simulink model "Main_with_GuiG"  (R2025b)
settings: Solver=VariableStepAuto  StartTime=0.0  StopTime=10.0  RelTol=1e-3
libraries: SignalEditorBlockLib x2, simulink x2, sharedTrackingLibrary x1, sim3dlib x1, uavsim3dlib x1, sensorgpslib x1, aerolibnav x1
settings Model: Creator=amirs  LastModifiedBy=amirs

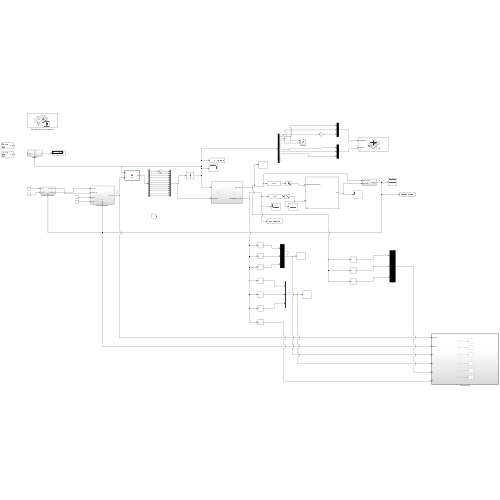
[thumbnail: Simulink's stored preview of the top-level diagram]
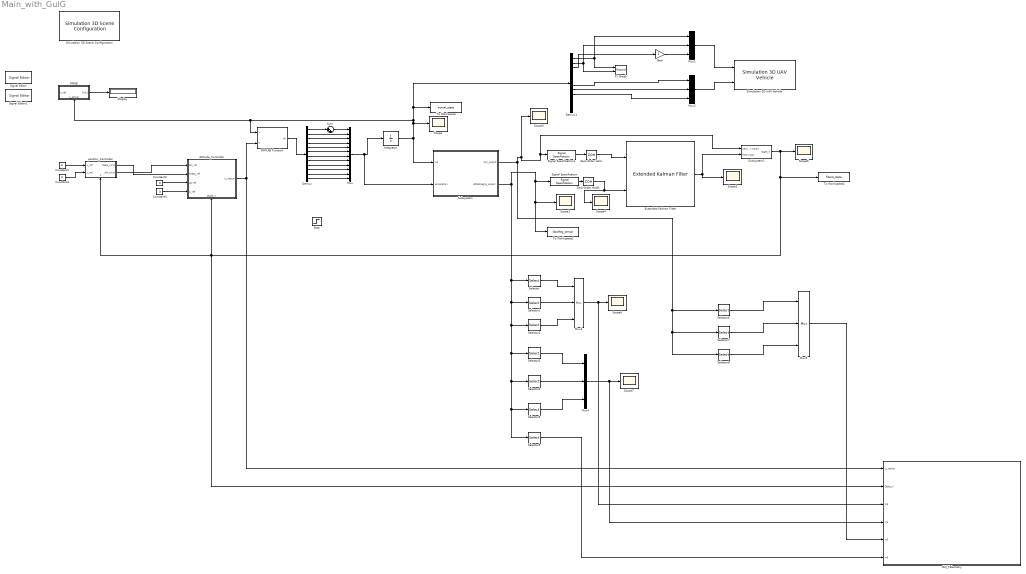
== system Main_with_GuiG ==
  Attitude_Controller : Subsystem
      settings: PortSchema="{\"entries\":[{\"content\":{\"sides\":[{\"content\":{\"connectorIds\":[\"In1\",\"In2\",\"In3\",\"In4\"]},\"type\":\"ConnectorPlacement.EquallySpacedRectSide\",\"uuid\":\"19f4eeea-d5cb-4ed7-9c59-67184399f9de\"},{\"content\":{\"connectorIds\":[\"Out1\"],\"side\":\"RIGHT\"},\"type\":\"ConnectorPlacement.EquallySpacedRectSide\",\"uuid\":\"b3f5ec5c-a38f-4295-9bcf-0fae3bfa674b\"},{\"content\":{\"side\":\"TOP\"},\"type\":\"ConnectorPlacement.EquallySpacedRectSide\",\"uuid\":\"2fc47e81-4ab5-4bbe-b029-56bfdcdb6174\"},{\"content\":{\"connectorIds\":[\"In5\"],\"side\":\"BOTTOM\"},\"type\":\"ConnectorPlacement.EquallySpacedRectSide\",\"uuid\":\"a7c3fd73-d82a-467d-bca9-1f7d01263d9c\"}]},\"type\":\"ConnectorPlacement.EquallySpacedConnector\",\"uuid\":\"700c1ad5-606a-4180-bf9f-c597a2a2a5d4\"}],\"packageUris\":[\"http://schema.mathworks.com/mf0/Connector/R2020b\"],\"version\":\"1.0\"}"
  Constant1 : Constant  Value=3
  Constant2 : Constant  Value=0
  Constant3 : Constant  Value=3
  Constant4 : Constant  Value=2
  Demux : Demux  Outputs=12
  Demux1 : Demux  Outputs=12
  Display : Display
  Extended Kalman Filter : sharedTrackingLibrary/Extended Kalman Filter  StateTransitionFcn=ekfStateTransition  HasStateTransitionJacobianFcn=off  HasAdditiveProcessNoise=Additive  ProcessNoise="[1e-5 1e-5 1e-5  1e-2 1e-2 1e-2  1.5e-6 1.5e-6 1.5e-6]"  HasTimeVaryingProcessNoise=off  HasStateTransitionFcnExtraArgument=1  InitialState=[0,0,0,0,0,0,0,0,0]  InitialStateCovariance=[6.25 6.25 0.04 2.5e-3 2.5e-3 2.5e-3 3e-3 3e-3 1.2e-3]  MeasurementFcn1=ekfMeasurement  HasMeasurementJacobianFcn1=off  HasMeasurementEnablePort1=off  HasAdditiveMeasurementNoise1=Additive  MeasurementNoise1="diag([6.25  7  0.04   2.5e-3  2.5e-3  2.5e-3   1.2e-3])"  HasTimeVaryingMeasurementNoise1=off  HasMeasurementFcnExtraArgument1=0  HasMeasurementWrapping1=off  MeasurementFcn2=ekfMeasTilt  HasMeasurementJacobianFcn2=off  HasMeasurementEnablePort2=off  HasAdditiveMeasurementNoise2=Additive  MeasurementNoise2=diag([2.5e-4 2.5e-4])  HasTimeVaryingMeasurementNoise2=off  HasMeasurementFcnExtraArgument2=0  HasMeasurementWrapping2=off  MeasurementFcn3=myMeasurementFcn  HasMeasurementJacobianFcn3=off  HasMeasurementEnablePort3=off  HasAdditiveMeasurementNoise3=Additive  MeasurementNoise3=1  HasTimeVaryingMeasurementNoise3=off  HasMeasurementFcnExtraArgument3=0  HasMeasurementWrapping3=off  MeasurementFcn4=myMeasurementFcn  HasMeasurementJacobianFcn4=off  HasMeasurementEnablePort4=off  HasAdditiveMeasurementNoise4=Additive  MeasurementNoise4=1  HasTimeVaryingMeasurementNoise4=off  HasMeasurementFcnExtraArgument4=0  HasMeasurementWrapping4=off  MeasurementFcn5=myMeasurementFcn  HasMeasurementJacobianFcn5=off  HasMeasurementEnablePort5=off  HasAdditiveMeasurementNoise5=Additive  MeasurementNoise5=1  HasTimeVaryingMeasurementNoise5=off  HasMeasurementFcnExtraArgument5=0  HasMeasurementWrapping5=off  EnableMultirate=on  StateTransitionFcnSampleTime=0.005  MeasurementFcn1SampleTime=0.1  MeasurementFcn2SampleTime=0.005  MeasurementFcn3SampleTime=1  MeasurementFcn4SampleTime=1  MeasurementFcn5SampleTime=1  UseCurrentEstimator=off  OutputStateCovariance=off  DataType=double  SampleTime=1  NumberOfMeasurements=1
  GUI_Telemetry : Subsystem  TreatAsAtomicUnit=on
  Gain : Gain
  Integrator : Integrator  InitialCondition=[0;0;0;0;0;0;0;0;0;0;0;0]
  MATLAB Function : MATLAB Function  TreatAsAtomicUnit=on
  Mux : Mux  Inputs=12
  Mux{1..5} (5 alike) : Mux  Inputs=3
  RMSE : Subsystem
      settings: PortSchema="{\"entries\":[{\"content\":{\"sides\":[{\"content\":{\"connectorIds\":[\"In1\"]},\"type\":\"ConnectorPlacement.EquallySpacedRectSide\",\"uuid\":\"5e07c89f-ef09-4b0a-bed5-e0d03eb8d545\"},{\"content\":{\"connectorIds\":[\"Out1\"],\"side\":\"RIGHT\"},\"type\":\"ConnectorPlacement.EquallySpacedRectSide\",\"uuid\":\"9156e923-85eb-42fc-9dec-5f08a3c9d42c\"},{\"content\":{\"side\":\"TOP\"},\"type\":\"ConnectorPlacement.EquallySpacedRectSide\",\"uuid\":\"e2ee007b-856b-4d03-8afd-b743321baf7d\"},{\"content\":{\"connectorIds\":[\"In2\"],\"side\":\"BOTTOM\"},\"type\":\"ConnectorPlacement.EquallySpacedRectSide\",\"uuid\":\"3aca7e9a-13ba-49c1-8015-1f7d41362bc4\"}]},\"type\":\"ConnectorPlacement.EquallySpacedConnector\",\"uuid\":\"905e6a99-45d0-4759-a1dd-bed499fabe76\"}],\"packageUris\":[\"http://schema.mathworks.com/mf0/Connector/R2020b\"],\"version\":\"1.0\"}"
  Scope{,1..7} (8 alike) : Scope
      Scope settings: ActiveDisplayYMinimum=-0.58911175900886825  ActiveDisplayYMaximum=5.302005831079815
      Scope1 settings: ActiveDisplayYMinimum=-13.326141979899816  ActiveDisplayYMaximum=19.254724347414861
      Scope2 settings: ActiveDisplayYMinimum=-0.53363237481390613  ActiveDisplayYMaximum=4.8026913733251559  DataLoggingVariableName=ScopeData2
      Scope3 settings: ActiveDisplayYMinimum=-7.8319587540170037  ActiveDisplayYMaximum=0.35536866604481165  DataLoggingVariableName=ScopeData5
      Scope4 settings: ActiveDisplayYMinimum=-7.5918797397091611  ActiveDisplayYMaximum=10.762543329699707  DataLoggingVariableName=ScopeData7
      Scope5 settings: ActiveDisplayYMinimum=-1.7341932188779878  ActiveDisplayYMaximum=7.0655008286033389  DataLoggingVariableName=ScopeData8
      Scope6 settings: ActiveDisplayYMinimum=-7.5918797397091611  ActiveDisplayYMaximum=10.762543329699707  DataLoggingVariableName=ScopeData10
      Scope7 settings: ActiveDisplayYMinimum=-7.5918797397091611  ActiveDisplayYMaximum=10.762543329699707  DataLoggingVariableName=ScopeData11
  Selector : Selector  InputPortWidth=7  IndexOptions=Index vector (dialog)  Indices=[1]  OutputSizes=1
  Selector1 : Selector  InputPortWidth=7  IndexOptions=Index vector (dialog)  Indices=[2]  OutputSizes=1
  Selector2 : Selector  InputPortWidth=7  IndexOptions=Index vector (dialog)  Indices=[3]  OutputSizes=1
  Selector3 : Selector  InputPortWidth=7  IndexOptions=Index vector (dialog)  Indices=[4]  OutputSizes=1
  Selector4 : Selector  InputPortWidth=7  IndexOptions=Index vector (dialog)  Indices=[5]  OutputSizes=1
  Selector5 : Selector  InputPortWidth=7  IndexOptions=Index vector (dialog)  Indices=[6]  OutputSizes=1
  Selector6 : Selector  InputPortWidth=6  IndexOptions=Index vector (dialog)  Indices=[1]  OutputSizes=1
  Selector7 : Selector  InputPortWidth=6  IndexOptions=Index vector (dialog)  Indices=[2]  OutputSizes=1
  Selector8 : Selector  InputPortWidth=6  IndexOptions=Index vector (dialog)  Indices=[3]  OutputSizes=1
  Selector9 : Selector  InputPortWidth=7  IndexOptions=Index vector (dialog)  Indices=[7]  OutputSizes=1
  Signal Editor : SignalEditorBlockLib/Signal Editor  FileName=squer.mat  ActiveScenario=Scenario  ActiveSignal=x_ref  IsBus=off  OutputBusObjectStr=Bus: BusObject  SampleTime=0  ZeroCross=off  OutputAfterFinalValue=Setting to zero  Unit=inherit  PreserveSignalName=on  ApplySigPropsToAllScenarios=on  ApplySigPropsToAllSignals=off  SignalPropertySource=Dialog parameters
  Signal Editor1 : SignalEditorBlockLib/Signal Editor  FileName=squer_y.mat  ActiveScenario=Scenario  ActiveSignal=y_ref  IsBus=off  OutputBusObjectStr=Bus: BusObject  SampleTime=0  ZeroCross=off  OutputAfterFinalValue=Setting to zero  Unit=inherit  PreserveSignalName=on  ApplySigPropsToAllScenarios=on  ApplySigPropsToAllSignals=off  SignalPropertySource=Dialog parameters
  Signal Specification : SignalSpecification  Dimensions=[7]
  Signal Specification1 : SignalSpecification
  Simulation 3D Scene Configuration : sim3dlib/Simulation 3D Scene Configuration  Priority=0  ProjectFormat=Default Scenes  SceneDesc=US city block  ProjectName=C:\Program Files\MATLAB\R2025b\toolbox\shared\sim3d_projects\automotive_project_windows\UE\WindowsNoEditor\VehicleSimulation.exe  ScenePath=/Game/Maps/USCityBlock  EnableOpenDRIVE=off  vehTagList={'Custom';'Scene Origin'}  vehTag=Scene Origin  AttachedCameraRelativeTranslation=[0 0 0]  FreeCameraDefaultInitialTranslation=[-6, 0, 2]  AttachedCameraRelativeRotation=[0 0 0]  FreeCameraDefaultInitialRotation=[0, -15, 0]  ViewpointName=Custom  FreeCameraInitialTranslation=[0, 0, 0]  ViewpointTranslation=[0, 0, 0]  FreeCameraInitialRotation=[0, 0, 0]  ViewpointRotation=[0, 0, 0]  OpVisEn=off  Ts=1/60  EnableWindow=on  EnableRemoteAccess=off  EnableWeather=off  SunAzimuth=90  SunAltitude=40.0  EnableGeospatialSun=off  Latitude=0  Longitude=0  Date=2023-01-01  Time=10:30:00  GeoTimeZone=-5.0  SunDaylightSaving=off  wind=1  clouds=10  EnableVolumetricClouds=off  CloudCoverage=0  CloudAltitude=6  fog=0  rain=0  RaindropsEffect=off  SnowDensity=0  EnableGeospatial=off  TilesetSource=Earth terrain  UseTrueOrigin=off  OriginHeight=200  OriginLatitude=40.744652  OriginLongitude=-73.988864  MapStyle=Aerial  AdditionalAssetIDs=[]  UseAdvancedSunSky=off  SolarTime=11  TimeZone=-5  Day=21  Month=9  Year=2022  UseDaylightSavingTime=on  DSTStartDay=10  DSTStartMonth=3  DSTEndDay=3  DSTEndMonth=11  DSTSwitchHour=2  sensorTag=MainCamera1  sensorId=1  sensorName=MainCamera1  mountLoc=Origin  offsetFlag=off  tmountOffset=[0, 0, 0]  rmountOffset=[0, 0, 0]  HorizontalResolution=1280  VerticalResolution=720  HorizontalFOV=60  mountPoint=[0 0 0]  mountOrientation=[0 0 0]  aMode=4  ID=1  GeoTrigger=Inactive  ViewNameList={'Custom'}  ViewTranslationList={'[0 0 0]'}  ViewRotationList={'[0 0 0]'}
      settings: LibrarySourceBlock=uavsim3dlib/Simulation 3D Scene Configuration
  Simulation 3D UAV Vehicle : uavsim3dlib/Simulation 3D UAV Vehicle  Priority=-1  Mesh=Quadrotor  MeshPath=/MathWorksUAVContent/UAVs/HexaRotorUAV/HexaRotor.HexaRotor  Color=Green  ActorName=SimulinkVehicle1  UseGlobalFrame=off  InitialTranslation=[0 0 0]  InitialRotation=[0 0 0]  InitialTranslationGlobal=[0 0 0]  InitialGeoOrigin=[0 0 0]  InitialRotationGlobal=[0 0 0]  SampleTime=-1  ActorType=SimulinkVehicle  ID=1  aMode=4  ActorTag=SimulinkVehicle1
  Step : Step  Time=25  After=0  SampleTime=0
  Subsystem : Subsystem
  Subsystem1 : Subsystem
  Sum : Sum  Inputs=|++
  To Workspace : ToWorkspace  VariableName=actual_state  SampleTime=-1
      settings: Save2DSignal=2-D array (concatenate along first dimension)
  To Workspace1 : ToWorkspace  VariableName=GpsMag_sensor  SampleTime=-1
      settings: Save2DSignal=2-D array (concatenate along first dimension)
  To Workspace2 : ToWorkspace  VariableName=filterd_state  SampleTime=-1
      settings: Save2DSignal=2-D array (concatenate along first dimension)
  XY Graph : Record  NumPorts=2.0  FileSettingsInternal="{\"entries\":[{\"content\":{\"excelSettings\":{\"content\":{},\"type\":\"Streamout.ExcelSettings\"},\"parquetSettings\":{\"content\":{},\"type\":\"Streamout.ParquetSettings\"}},\"type\":\"Streamout.FileSettingStorage\",\"uuid\":\"\"}],\"packageUris\":[\"http:\\/\\/schema.mathworks.com\\/mf0\\/streamout_blocks\\/R2020a\"],\"version\":\"1.0\"}"  FrameSettings=[0, 0]  Layout=[1 1]  SignalsInternal="{\"entries\":[{\"content\":{\"signals\":[{\"content\":{\"blockPath\":[],\"dimensions\":[1],\"domain\":\"\",\"lineColor\":\"#64d413\",\"lineWidth\":2,\"port\":1,\"sid\":[\"\"],\"signalID\":1,\"signalName\":\"Demux1:1\"},\"type\":\"RecordBlkView.Signal\",\"uuid\":\"\"},{\"content\":{\"blockPath\":[],\"dimensions\":[1],\"domain\":\"\",\"lineColor\":\"#ff13a6\",\"lineWidth\":2,\"port\":2,\"sid\":[\"\"],\"signalID\":2,\"signalName\":\"Demux1:2\"},\"type\":\"RecordBlkView.Signal\",\"uuid\":\"\"}]},\"type\":\"RecordBlkView.InputSignals\",\"uuid\":\"\"}],\"packageUris\":[\"http:\\/\\/schema.mathworks.com\\/mf0\\/streamout_blocks\\/R2020a\"],\"version\":\"1.0\"}"  VisualizationBindings="{\"xyplotplugin\":{\"info\":[{\"series\":[],\"subplotID\":1}]}}"  CompatibilityTag=XY
  Zero-Order Hold : ZeroOrderHold  SampleTime=0.005
  Zero-Order Hold1 : ZeroOrderHold  SampleTime=0.1
  position_Controller : Subsystem
      settings: PortSchema="{\"entries\":[{\"content\":{\"sides\":[{\"content\":{\"connectorIds\":[\"In1\",\"In2\"]},\"type\":\"ConnectorPlacement.EquallySpacedRectSide\",\"uuid\":\"b3fdc6c0-3d6b-4fed-ba04-72ee8971ce33\"},{\"content\":{\"connectorIds\":[\"Out1\",\"Out2\"],\"side\":\"RIGHT\"},\"type\":\"ConnectorPlacement.EquallySpacedRectSide\",\"uuid\":\"c5fff90f-3f0d-4e66-bfd3-42639056edf5\"},{\"content\":{\"side\":\"TOP\"},\"type\":\"ConnectorPlacement.EquallySpacedRectSide\",\"uuid\":\"29c618c7-b581-4d0e-90c8-5996712070e8\"},{\"content\":{\"connectorIds\":[\"In3\"],\"side\":\"BOTTOM\"},\"type\":\"ConnectorPlacement.EquallySpacedRectSide\",\"uuid\":\"80cb8360-5186-4b4a-b3bf-580e229b7937\"}]},\"type\":\"ConnectorPlacement.EquallySpacedConnector\",\"uuid\":\"86696893-c9ee-41ff-bf75-cf6f558ac07e\"}],\"packageUris\":[\"http://schema.mathworks.com/mf0/Connector/R2020b\"],\"version\":\"1.0\"}"
  wires:
  Demux/12 -> Mux/12
  Demux/6 -> Mux/6
  Sum/1 -> Mux/1
  Mux/1 -> Subsystem/2(accleration), Integrator/1
  Demux/1 -> Sum/1
  RMSE/1(Out1) -> Display/1
  Gain/1 -> Mux1/3
  position_Controller/1(theta_cmd) -> Attitude_Controller/2(Theta_ref)
  Extended Kalman Filter/1 -> Subsystem1/2(filter input), Scope2/1
  Demux/5 -> Mux/5
  Subsystem/2(GPS&Magno_output) -> To Workspace1/1, Scope1/1, Signal Specification/1, Selector4/1, Selector9/1, Selector5/1, Selector3/1, Selector2/1, Selector1/1, Selector/1
  Demux/4 -> Mux/4
  Integrator/1 -> Subsystem/1(In1), Scope/1, To Workspace/1, Demux1/1, MATLAB Function/1(X), RMSE/2(x_actual)
  Demux/9 -> Mux/9
  Demux/11 -> Mux/11
  Zero-Order Hold/1 -> Extended Kalman Filter/1
  Demux1/2 -> XY Graph/2, Mux1/2
  Subsystem1/1(State_X) -> To Workspace2/1, GUI_Telemetry/2(State_X), position_Controller/3(X), Attitude_Controller/5(State_X), Scope5/1
  Demux/3 -> Mux/3
  Demux/2 -> Mux/2
  Demux1/7 -> Mux2/1
  Constant1/1 -> position_Controller/1(x_ref)
  position_Controller/2(phi_cmd) -> Attitude_Controller/1(phi_ref)
  Demux1/8 -> Mux2/2
  Demux1/9 -> Mux2/3
  Signal Specification/1 -> Zero-Order Hold1/1
  Constant3/1 -> Attitude_Controller/4(Z_ref)
  Demux1/1 -> Mux1/1, XY Graph/1
  Zero-Order Hold1/1 -> Extended Kalman Filter/2, Scope4/1
  Demux1/3 -> Gain/1
  Demux/8 -> Mux/8
  Mux2/1 -> Simulation 3D UAV Vehicle/2
  Demux/10 -> Mux/10
  Signal Specification1/1 -> Zero-Order Hold/1
  Demux/7 -> Mux/7
  Attitude_Controller/1(U_vector) -> MATLAB Function/2(U), GUI_Telemetry/1(U_vector)
  MATLAB Function/1(dX) -> Demux/1
  Constant2/1 -> Attitude_Controller/3(psi ref)
  Mux1/1 -> Simulation 3D UAV Vehicle/1
  Constant4/1 -> position_Controller/2(y_ref)
  Selector/1 -> Mux3/1
  Selector1/1 -> Mux3/2
  Selector2/1 -> Mux3/3
  Mux3/1 -> GUI_Telemetry/3(In3), Scope6/1
  Selector3/1 -> Mux4/1
  Selector4/1 -> Mux4/2
  Selector5/1 -> Mux4/3
  Mux4/1 -> GUI_Telemetry/4(In4), Scope7/1
  Subsystem/1(IMU_output) -> Subsystem1/1(sensor input1), Signal Specification1/1, Scope3/1, Selector8/1, Selector7/1, Selector6/1
  Selector7/1 -> Mux5/2
  Selector8/1 -> Mux5/3
  Selector6/1 -> Mux5/1
  Mux5/1 -> GUI_Telemetry/5(In5)
  Selector9/1 -> GUI_Telemetry/6(In6)

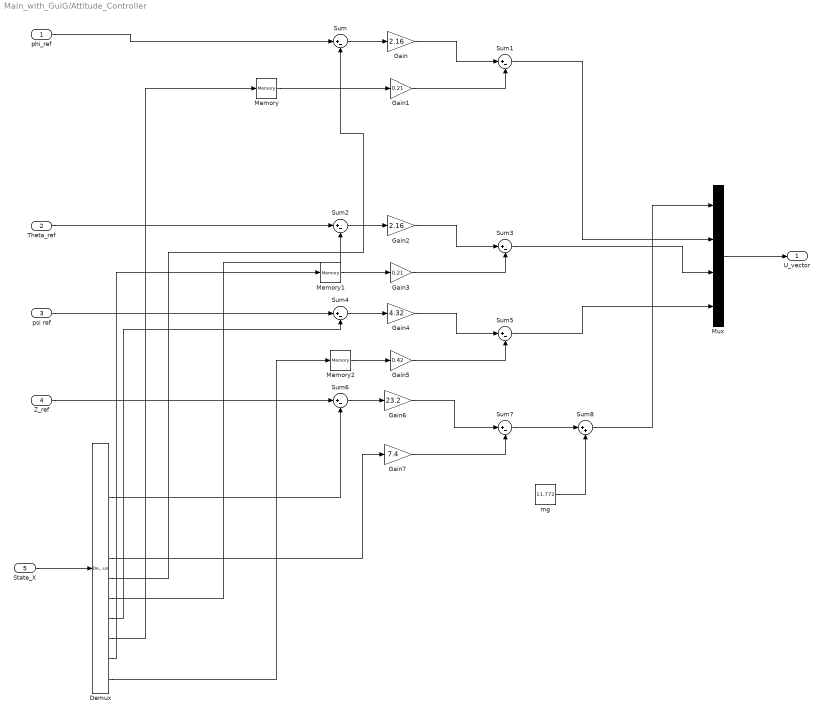
== system Main_with_GuiG/Attitude_Controller ==
  phi_ref : Inport
  Theta_ref : Inport  Port=2
  psi ref : Inport  Port=3
  Z_ref : Inport  Port=4
  State_X : Inport  Port=5
  Demux : Demux  Outputs=12
  Gain : Gain  Gain=2.16
  Gain1 : Gain  Gain=0.21
  Gain2 : Gain  Gain=2.16
  Gain3 : Gain  Gain=0.21
  Gain4 : Gain  Gain=4.32
  Gain5 : Gain  Gain=0.42
  Gain6 : Gain  Gain=23.2
  Gain7 : Gain  Gain=7.4
  Memory : Memory
  Memory1 : Memory
  Memory2 : Memory
  Mux : Mux
  Sum{,1..7} (8 alike) : Sum  Inputs=|+-
  Sum8 : Sum  Inputs=|++
  mg : Constant  Value=11.772
  U_vector : Outport
  wires:
  State_X/1 -> Demux/1
  phi_ref/1 -> Sum/1
  Demux/7 -> Sum/2
  Sum/1 -> Gain/1
  Gain/1 -> Sum1/1
  Gain1/1 -> Sum1/2
  Gain3/1 -> Sum3/2
  Gain2/1 -> Sum3/1
  Sum2/1 -> Gain2/1
  Theta_ref/1 -> Sum2/1
  Demux/8 -> Sum2/2
  Gain5/1 -> Sum5/2
  Gain4/1 -> Sum5/1
  Sum4/1 -> Gain4/1
  psi ref/1 -> Sum4/1
  Demux/9 -> Sum4/2
  Z_ref/1 -> Sum6/1
  Demux/3 -> Sum6/2
  Sum6/1 -> Gain6/1
  Demux/6 -> Gain7/1
  Gain6/1 -> Sum7/1
  Gain7/1 -> Sum7/2
  Sum7/1 -> Sum8/1
  mg/1 -> Sum8/2
  Sum8/1 -> Mux/1
  Sum1/1 -> Mux/2
  Sum3/1 -> Mux/3
  Sum5/1 -> Mux/4
  Mux/1 -> U_vector/1
  Memory/1 -> Gain1/1
  Demux/10 -> Memory/1
  Memory1/1 -> Gain3/1
  Demux/11 -> Memory1/1
  Memory2/1 -> Gain5/1
  Demux/12 -> Memory2/1

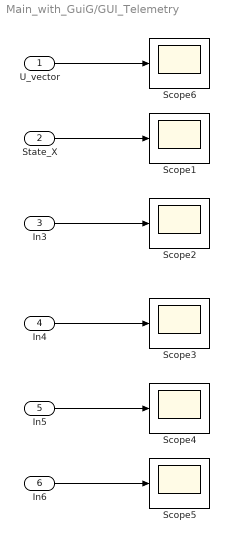
== system Main_with_GuiG/GUI_Telemetry ==
  U_vector : Inport
  State_X : Inport  Port=2
  In3 : Inport  Port=3
  In4 : Inport  Port=4
  In5 : Inport  Port=5
  In6 : Inport  Port=6
  Scope{1..6} (6 alike) : Scope
      Scope1 settings: ActiveDisplayYMinimum=-7.5918797397091611  ActiveDisplayYMaximum=10.762543329699707  DataLoggingVariableName=ScopeData13
      Scope2 settings: ActiveDisplayYMinimum=-7.5918797397091611  ActiveDisplayYMaximum=10.762543329699707  DataLoggingVariableName=ScopeData14
      Scope3 settings: ActiveDisplayYMinimum=-7.5918797397091611  ActiveDisplayYMaximum=10.762543329699707  DataLoggingVariableName=ScopeData15
      Scope4 settings: ActiveDisplayYMinimum=-7.5918797397091611  ActiveDisplayYMaximum=10.762543329699707  DataLoggingVariableName=ScopeData16
      Scope5 settings: ActiveDisplayYMinimum=-7.5918797397091611  ActiveDisplayYMaximum=10.762543329699707  DataLoggingVariableName=ScopeData17
      Scope6 settings: ActiveDisplayYMinimum=-7.5918797397091611  ActiveDisplayYMaximum=10.762543329699707  DataLoggingVariableName=ScopeData12
  wires:
  U_vector/1 -> Scope6/1
  State_X/1 -> Scope1/1
  In3/1 -> Scope2/1
  In4/1 -> Scope3/1
  In5/1 -> Scope4/1
  In6/1 -> Scope5/1

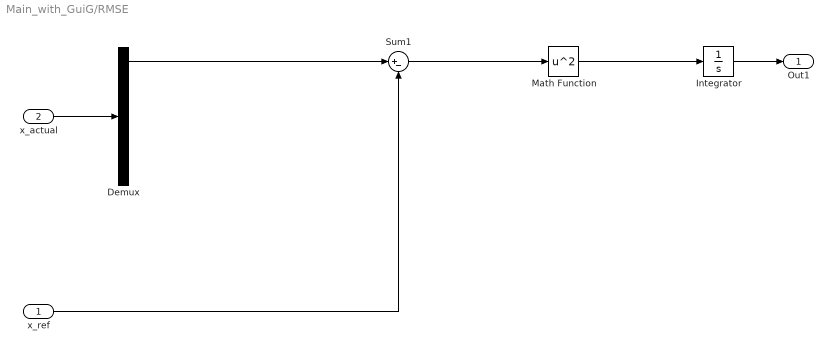
== system Main_with_GuiG/RMSE ==
  x_ref : Inport
  x_actual : Inport  Port=2
  Demux : Demux  Outputs=12
  Integrator : Integrator
  Math Function : Math  Operator=square
  Sum1 : Sum  Inputs=|+-
  Out1 : Outport
  wires:
  x_actual/1 -> Demux/1
  x_ref/1 -> Sum1/2
  Demux/1 -> Sum1/1
  Sum1/1 -> Math Function/1
  Math Function/1 -> Integrator/1
  Integrator/1 -> Out1/1

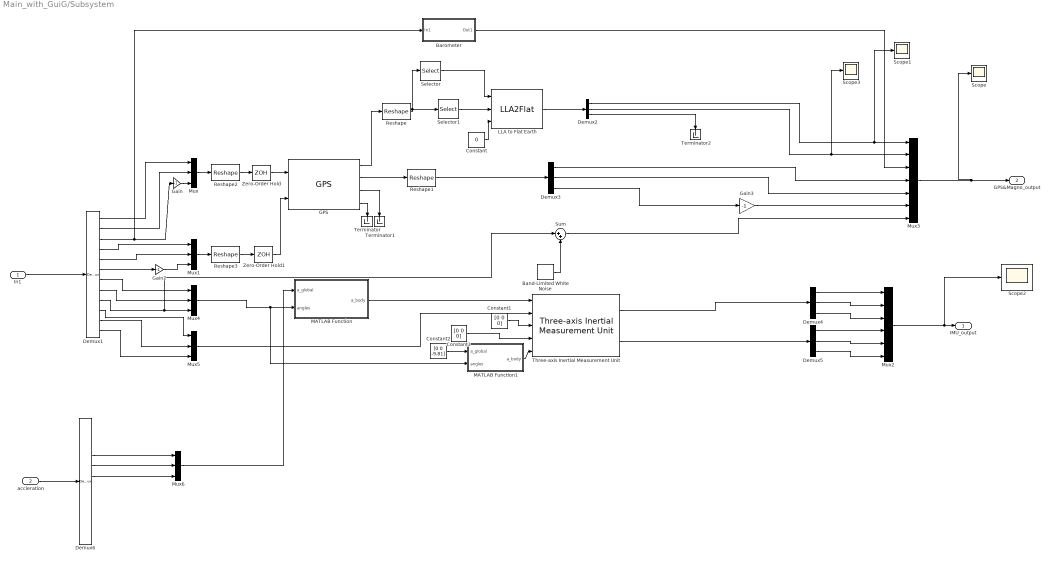
== system Main_with_GuiG/Subsystem ==
  In1 : Inport
  accleration : Inport  Port=2
  Band-Limited White Noise : simulink/Sources/Band-Limited White Noise  Cov=1.2e-4  Ts=0.1  seed=[23341]
  Barometer : Subsystem
  Constant : Constant  Value=0
  Constant1 : Constant  Value=[0 0 0]
  Constant2 : Constant  Value=[0 0 -9.81]
  Constant3 : Constant  Value=[0 0 0]
  Demux1 : Demux  Outputs=12
  Demux{2..5} (4 alike) : Demux  Outputs=3
  Demux6 : Demux  Outputs=12
  GPS : sensorgpslib/GPS  DispRefFrame=NED  PositionInputFormat=Local  ReferenceLocation=[ 0, 0, 0 ]  HorizontalPositionAccuracy=2.5  VerticalPositionAccuracy=5  VelocityAccuracy=0.05  DecayFactor=0  SeedDouble=67  SimulateUsing=Interpreted execution
      settings: LibrarySourceBlock=uavsimlib/GPS
  Gain : Gain  Gain=-1
  Gain2 : Gain  Gain=-1
  Gain3 : Gain  Gain=-1
  LLA to Flat Earth : LLA2Flat  LL0=[0 0]
  MATLAB Function : MATLAB Function  TreatAsAtomicUnit=on
  MATLAB Function1 : MATLAB Function  TreatAsAtomicUnit=on
  Mux{,1,4..6} (5 alike) : Mux  Inputs=3
  Mux2 : Mux  Inputs=6
  Mux3 : Mux  Inputs=7
  Reshape : Reshape  OutputDimensionality=Column vector (2-D)
  Reshape1 : Reshape
  Reshape2 : Reshape  OutputDimensionality=Row vector (2-D)
  Reshape3 : Reshape  OutputDimensionality=Row vector (2-D)
  Scope{,1..3} (4 alike) : Scope
      Scope settings: ActiveDisplayYMinimum=-1.2523614527770178E+6  ActiveDisplayYMaximum=139169.27196179639  DataLoggingVariableName=ScopeData3
      Scope1 settings: ActiveDisplayYMinimum=-13.357949302469024  ActiveDisplayYMaximum=19.483647605831496  DataLoggingVariableName=ScopeData4
      Scope2 settings: ActiveDisplayYMinimum=-6.4871029575674033  ActiveDisplayYMaximum=8.1253486671858823  DataLoggingVariableName=ScopeData6
      Scope3 settings: ActiveDisplayYMinimum=-16.905633944081533  ActiveDisplayYMaximum=17.427001489825049  DataLoggingVariableName=ScopeData9
  Selector : Selector  NumberOfDimensions=2  InputPortWidth=3  IndexOptions=Index vector (dialog),Select all  Indices=[1 2],1  OutputSizes=1,1
  Selector1 : Selector  NumberOfDimensions=2  InputPortWidth=3  IndexOptions=Index vector (dialog),Select all  Indices=3,1  OutputSizes=1,1
  Sum : Sum  Inputs=|++
  Terminator : Terminator
  Terminator1 : Terminator
  Terminator2 : Terminator
  Three-axis Inertial Measurement Unit : aerolibnav/Three-axis Inertial Measurement Unit  units=Metric (MKS)  imu=[0 0 0]  i_Ts=0  dtype_a=on  w_a=190  z_a=0.707  a_sf_cc=[1 0 0; 0 1 0; 0 0 1]  a_bias=[0 0 0]  a_sat="[-inf  -inf  -inf  inf inf inf]"  dtype_g=on  w_g=190  z_g=0.707  g_sf_cc=[1 0 0; 0 1 0; 0 0 1]  g_bias=[0 0 0]  g_sens=[0 0 0]  g_sat="[-inf  -inf  -inf  inf inf inf]"  i_rand=on  i_seeds=[23093 23094 23095 23096 23097 23098]  i_pow="[8.6e-6  8.6e-6  8.6e-6   3.1e-8  3.1e-8  3.1e-8]"
  Zero-Order Hold : ZeroOrderHold  SampleTime=-1
  Zero-Order Hold1 : ZeroOrderHold  SampleTime=-1
  IMU_output : Outport
  GPS&Magno_output : Outport  Port=2
  wires:
  In1/1 -> Demux1/1
  Demux1/1 -> Mux/1
  Demux1/2 -> Mux/2
  Demux1/4 -> Mux1/1
  Demux1/5 -> Mux1/2
  Constant/1 -> LLA to Flat Earth/3
  LLA to Flat Earth/1 -> Demux2/1
  GPS/4 -> Terminator/1
  GPS/3 -> Terminator1/1
  Demux1/7 -> Mux4/1
  Demux1/8 -> Mux4/2
  Mux4/1 -> MATLAB Function1/2(angles), MATLAB Function/2(angles)
  MATLAB Function/1(a_body) -> Three-axis Inertial Measurement Unit/1
  Demux1/10 -> Mux5/1
  Demux1/11 -> Mux5/2
  Demux1/12 -> Mux5/3
  Mux5/1 -> Three-axis Inertial Measurement Unit/2
  Constant1/1 -> Three-axis Inertial Measurement Unit/3
  Gain/1 -> Mux/3
  Demux1/3 -> Barometer/1(In1), Gain/1
  Demux2/3 -> Terminator2/1
  Constant2/1 -> MATLAB Function1/1(a_global)
  MATLAB Function1/1(a_body) -> Three-axis Inertial Measurement Unit/5
  Three-axis Inertial Measurement Unit/2 -> Demux5/1
  Demux1/9 -> Mux4/3, Sum/1
  Demux1/6 -> Gain2/1
  Gain2/1 -> Mux1/3
  Demux3/3 -> Gain3/1
  accleration/1 -> Demux6/1
  Demux6/4 -> Mux6/1
  Demux6/5 -> Mux6/2
  Demux6/6 -> Mux6/3
  Mux6/1 -> MATLAB Function/1(a_global)
  Three-axis Inertial Measurement Unit/1 -> Demux4/1
  GPS/1 -> Reshape/1
  Reshape/1 -> Selector/1, Selector1/1
  Selector/1 -> LLA to Flat Earth/1
  Selector1/1 -> LLA to Flat Earth/2
  GPS/2 -> Reshape1/1
  Reshape1/1 -> Demux3/1
  Mux/1 -> Reshape2/1
  Mux1/1 -> Reshape3/1
  Constant3/1 -> Three-axis Inertial Measurement Unit/4
  Reshape2/1 -> Zero-Order Hold/1
  Zero-Order Hold/1 -> GPS/1
  Reshape3/1 -> Zero-Order Hold1/1
  Zero-Order Hold1/1 -> GPS/2
  Band-Limited White Noise/1 -> Sum/2
  Demux4/1 -> Mux2/1
  Demux4/2 -> Mux2/2
  Demux4/3 -> Mux2/3
  Demux5/1 -> Mux2/4
  Demux5/2 -> Mux2/5
  Demux5/3 -> Mux2/6
  Mux2/1 -> Scope2/1, IMU_output/1
  Demux2/1 -> Mux3/1, Scope1/1
  Demux2/2 -> Mux3/2, Scope3/1
  Barometer/1(Out1) -> Mux3/3
  Demux3/1 -> Mux3/4
  Demux3/2 -> Mux3/5
  Gain3/1 -> Mux3/6
  Sum/1 -> Mux3/7
  Mux3/1 -> Scope/1, GPS&Magno_output/1

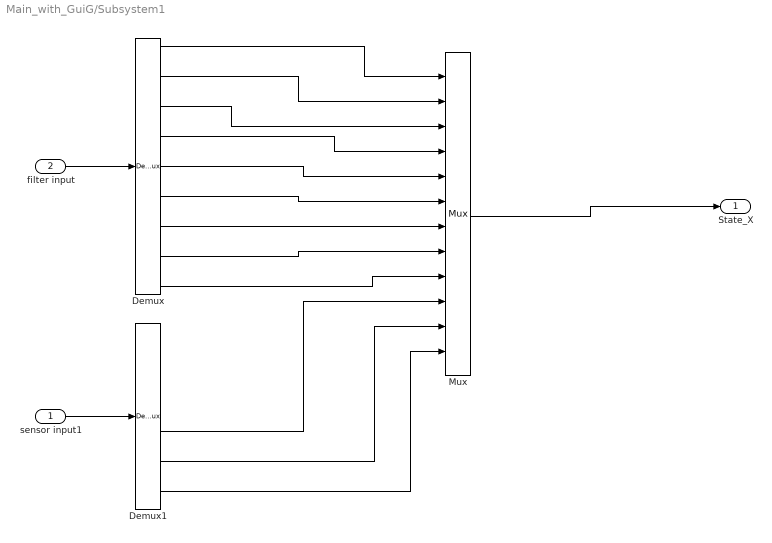
== system Main_with_GuiG/Subsystem1 ==
  sensor input1 : Inport
  filter input : Inport  Port=2
  Demux : Demux  Outputs=9
  Demux1 : Demux  Outputs=6
  Mux : Mux  Inputs=12
  State_X : Outport
  wires:
  filter input/1 -> Demux/1
  sensor input1/1 -> Demux1/1
  Demux/1 -> Mux/1
  Demux/2 -> Mux/2
  Demux/3 -> Mux/3
  Demux/4 -> Mux/4
  Demux/5 -> Mux/5
  Demux/6 -> Mux/6
  Demux/7 -> Mux/7
  Demux/8 -> Mux/8
  Demux/9 -> Mux/9
  Demux1/4 -> Mux/10
  Demux1/5 -> Mux/11
  Demux1/6 -> Mux/12
  Mux/1 -> State_X/1

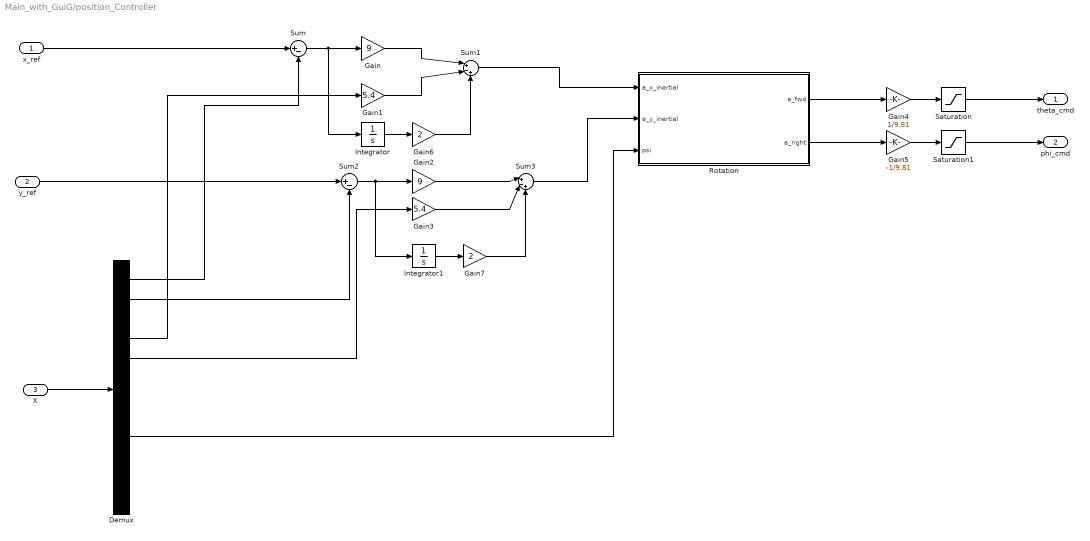
== system Main_with_GuiG/position_Controller ==
  x_ref : Inport
  y_ref : Inport  Port=2
  X : Inport  Port=3
  Demux : Demux  Outputs=12
  Gain : Gain  Gain=9
  Gain1 : Gain  Gain=5.4
  Gain2 : Gain  Gain=9
  Gain3 : Gain  Gain=5.4
  Gain4 : Gain  Gain=1/9.81
  Gain5 : Gain  Gain=-1/9.81
  Gain6 : Gain  Gain=2
  Gain7 : Gain  Gain=2
  Integrator : Integrator  LimitOutput=on  UpperSaturationLimit=5  LowerSaturationLimit=-5
  Integrator1 : Integrator  LimitOutput=on  UpperSaturationLimit=5  LowerSaturationLimit=-5
  Rotation : Subsystem
  Saturation : Saturate  UpperLimit=0.2  LowerLimit=-0.2
  Saturation1 : Saturate  UpperLimit=0.2  LowerLimit=-0.2
  Sum : Sum  Inputs=|+-
  Sum1 : Sum  Inputs=|+-+
  Sum2 : Sum  Inputs=|+-
  Sum3 : Sum  Inputs=|+-+
  theta_cmd : Outport
  phi_cmd : Outport  Port=2
  wires:
  X/1 -> Demux/1
  x_ref/1 -> Sum/1
  Demux/1 -> Sum/2
  Sum/1 -> Integrator/1, Gain/1
  Demux/4 -> Gain1/1
  Gain/1 -> Sum1/1
  Gain1/1 -> Sum1/2
  Gain3/1 -> Sum3/2
  Gain2/1 -> Sum3/1
  Sum2/1 -> Integrator1/1, Gain2/1
  y_ref/1 -> Sum2/1
  Demux/2 -> Sum2/2
  Demux/5 -> Gain3/1
  Sum3/1 -> Rotation/2(a_y_inertial)
  Demux/9 -> Rotation/3(psi)
  Rotation/1(a_fwd) -> Gain4/1
  Gain4/1 -> Saturation/1
  Saturation/1 -> theta_cmd/1
  Rotation/2(a_right) -> Gain5/1
  Gain5/1 -> Saturation1/1
  Saturation1/1 -> phi_cmd/1
  Sum1/1 -> Rotation/1(a_x_inertial)
  Integrator/1 -> Gain6/1
  Gain6/1 -> Sum1/3
  Integrator1/1 -> Gain7/1
  Gain7/1 -> Sum3/3

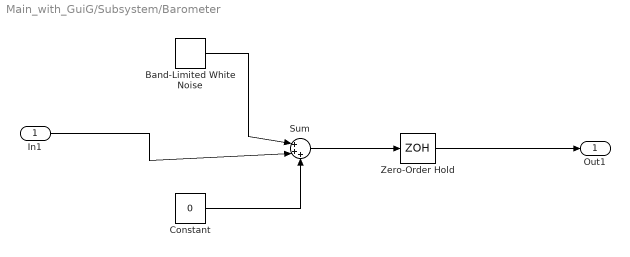
== system Main_with_GuiG/Subsystem/Barometer ==
  In1 : Inport
  Band-Limited White Noise : simulink/Sources/Band-Limited White Noise  Cov=[4.3e-5]  Ts=0.1  seed=[23341]
  Constant : Constant  Value=0
  Sum : Sum  Inputs=|+++
  Zero-Order Hold : ZeroOrderHold  SampleTime=-1
  Out1 : Outport
  wires:
  In1/1 -> Sum/2
  Sum/1 -> Zero-Order Hold/1
  Zero-Order Hold/1 -> Out1/1
  Band-Limited White Noise/1 -> Sum/1
  Constant/1 -> Sum/3

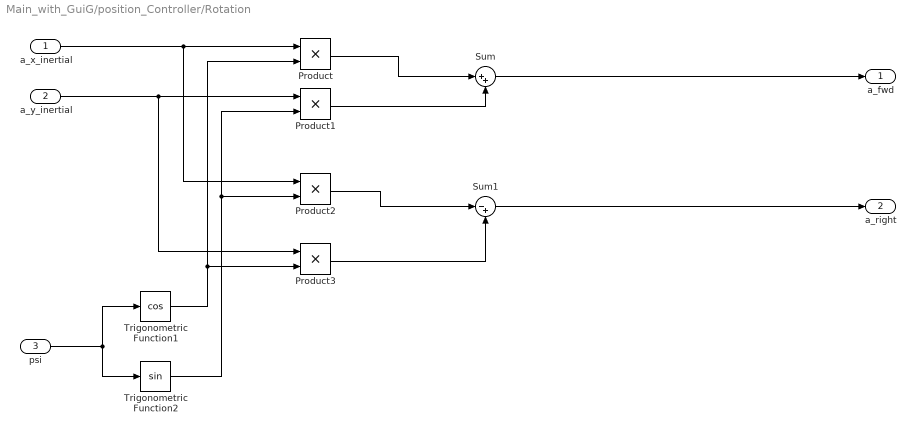
== system Main_with_GuiG/position_Controller/Rotation ==
  a_x_inertial : Inport
  a_y_inertial : Inport  Port=2
  psi : Inport  Port=3
  Product{,1..3} (4 alike) : Product
  Sum : Sum  Inputs=|++
  Sum1 : Sum  Inputs=|-+
  Trigonometric Function1 : Trigonometry  Operator=cos
  Trigonometric Function2 : Trigonometry
  a_fwd : Outport
  a_right : Outport  Port=2
  wires:
  psi/1 -> Trigonometric Function2/1, Trigonometric Function1/1
  a_x_inertial/1 -> Product2/1, Product/1
  Trigonometric Function1/1 -> Product3/2, Product/2
  a_y_inertial/1 -> Product3/1, Product1/1
  Trigonometric Function2/1 -> Product2/2, Product1/2
  Product/1 -> Sum/1
  Product1/1 -> Sum/2
  Sum/1 -> a_fwd/1
  Product2/1 -> Sum1/1
  Product3/1 -> Sum1/2
  Sum1/1 -> a_right/1

== matlab function Main_with_GuiG/MATLAB Function ==
  data: X input; dX output; U input
function dX=fcn(X,U)
        m= 1.2;
        g=9.81;
        Ixx=0.01;Iyy=0.01;Izz=0.02;
        phi=X(7);theta=X(8);psi=X(9);
        p = X(10);q=X(11);r=X(12);
        U1=U(1);U2=U(2);U3=U(3);U4=U(4);

        % Rotational Dyanamics:
        p_dot = (U2-(Izz-Iyy)*q*r)/Ixx;
        q_dot = (U3-(Ixx-Izz)*p*r)/Iyy;
        r_dot = (U4-(Iyy-Ixx)*p*q)/Izz;

        % 
        phi_dot= p + q*sin(phi)*tan(theta) + r*cos(phi)*tan(theta);
        theta_dot = q*cos(phi)-r*sin(phi);
        psi_dot = q*sin(phi)/cos(theta) + r*cos(phi)/cos(theta);

        % Translational
        ax = (U1/m)*(cos(phi)*sin(theta)*cos(psi) + sin(phi)*sin(psi));
        ay = (U1/m)*(cos(phi)*sin(theta)*sin(psi)- sin(phi)*cos(psi));
        az = (-1*g) + (U1/m)*(cos(phi)*cos(theta));

        dX = [X(4);X(5);X(6);ax;ay;az;phi_dot;theta_dot;psi_dot;p_dot;q_dot;r_dot];
end

== matlab function Main_with_GuiG/Subsystem/MATLAB Function1 ==
  data: a_global input; a_body output; angles input
function a_body = global_to_body(a_global, angles)
    % angles = [roll, pitch, yaw] in radians
    phi = angles(1);
    theta = angles(2);
    psi = angles(3);

    % Define the standard Z-Y-X rotation matrices
    R_z = [cos(psi) -sin(psi) 0; sin(psi) cos(psi) 0; 0 0 1];
    R_y = [cos(theta) 0 sin(theta); 0 1 0; -sin(theta) 0 cos(theta)];
    R_x = [1 0 0; 0 cos(phi) -sin(phi); 0 sin(phi) cos(phi)];

    % Multiply them to get the complete Body-to-Global matrix
    R_bg = R_z * R_y * R_x;
    
    % The Global-to-Body matrix is simply the transpose (inverse)
    R_gb = transpose(R_bg);

    % Rotate the global acceleration vector into the body frame
    a_body = R_gb * a_global;
end

== matlab function Main_with_GuiG/Subsystem/MATLAB Function ==
  data: a_global input; a_body output; angles input
function a_body = global_to_body(a_global, angles)
    % angles = [roll, pitch, yaw] in radians
    phi = angles(1);
    theta = angles(2);
    psi = angles(3);

    % Define the standard Z-Y-X rotation matrices
    R_z = [cos(psi) -sin(psi) 0; sin(psi) cos(psi) 0; 0 0 1];
    R_y = [cos(theta) 0 sin(theta); 0 1 0; -sin(theta) 0 cos(theta)];
    R_x = [1 0 0; 0 cos(phi) -sin(phi); 0 sin(phi) cos(phi)];

    % Multiply them to get the complete Body-to-Global matrix
    R_bg = R_z * R_y * R_x;
    
    % The Global-to-Body matrix is simply the transpose (inverse)
    R_gb = transpose(R_bg);

    % Rotate the global acceleration vector into the body frame
    a_body = R_gb * a_global;
end
